simulink model "integrated_controller_scenario3"  (R2021a)
settings: Solver=VariableStepAuto  StartTime=0.0  StopTime=50  RelTol=1e-3
values from neighbouring files (symbols this model uses):
  Cf = 155494.663    [integrated_controller_init.m]    (also in integrated_controller_init_q3.m; integrated_controller_init_q4.m; integrated_controller_init_q5.m; integrated_controller_init_q6_MRM.m)
  Cr = 1554494.663    [integrated_controller_init.m]    (also in integrated_controller_init_q3.m; integrated_controller_init_q4.m; integrated_controller_init_q5.m; integrated_controller_init_q6_MRM.m)
  Iz = 1436.24    [integrated_controller_init.m]    (also in integrated_controller_init_q3.m; integrated_controller_init_q4.m; integrated_controller_init_q5.m; integrated_controller_init_q6_MRM.m)
  L = 3.5    [alc_pathplanning.m]    (also in integrated_controller_init.m = 4.7; integrated_controller_init_q3.m = 4.7; integrated_controller_init_q4.m = 4.7; integrated_controller_init_q5.m = 4.7)
  ld = 10    [integrated_controller_init.m]    (also in integrated_controller_init_q3.m; integrated_controller_init_q4.m; integrated_controller_init_q5.m; integrated_controller_init_q6_MRM.m)
  lf = 1.165    [integrated_controller_init.m]    (also in integrated_controller_init_q3.m; integrated_controller_init_q4.m; integrated_controller_init_q5.m; integrated_controller_init_q6_MRM.m)
  lr = 1.165    [integrated_controller_init.m]    (also in integrated_controller_init_q3.m; integrated_controller_init_q4.m; integrated_controller_init_q5.m; integrated_controller_init_q6_MRM.m)
  m = 1140    [integrated_controller_init.m]    (also in integrated_controller_init_q3.m; integrated_controller_init_q4.m; integrated_controller_init_q5.m; integrated_controller_init_q6_MRM.m)
  md = get_curvature(Vx,yaw_rate_pose,tRef')    [integrated_controller_init.m]    (also in integrated_controller_init_q3.m; integrated_controller_init_q4.m; integrated_controller_init_q5.m; integrated_controller_init_q6_MRM.m)
  Ts = 0.1    [integrated_controller_init.m]    (also in integrated_controller_init_q3.m; integrated_controller_init_q4.m; integrated_controller_init_q5.m; integrated_controller_init_q6_MRM.m)
  V_initial = 15    [integrated_controller_init.m]    (also in integrated_controller_init_q3.m = 11; integrated_controller_init_q4.m = 25; integrated_controller_init_q5.m; integrated_controller_init_q6_MRM.m)
  Vx = a(2) + 2*a(3)*t + 3*a(4)*t.^2 +4*a(5)*t.^3+ a(6)*t.^4    [alc_pathplanning.m]    (also in integrated_controller_init.m = 18; integrated_controller_init_q3.m = 20; integrated_controller_init_q4.m = 25; integrated_controller_init_q5.m = 15)
  xRef = X_ref    [alc_pathplanning.m]    (also in integrated_controller_init.m = path.xRef; integrated_controller_init_q3.m = path.xRef; integrated_controller_init_q4.m = path.xRef; integrated_controller_init_q5.m = refPose(1,:))
  yRef = Y_ref    [alc_pathplanning.m]    (also in integrated_controller_init.m = path.yRef; integrated_controller_init_q3.m = path.yRef; integrated_controller_init_q4.m = path.yRef; integrated_controller_init_q5.m = refPose(2,:))
undefined symbols (not defined in the file or in its folder): sigbuilder_block
libraries: pid_lib x2, mpcadaslib x1, robotalgslib x1, autolibshared x1
settings Model: Creator=anime  LastModifiedBy=srini
settings SolverCC: AlgebraicLoopSolver=TrustRegion
settings DebuggingCC: SFMachineParentedDataDiag=warning

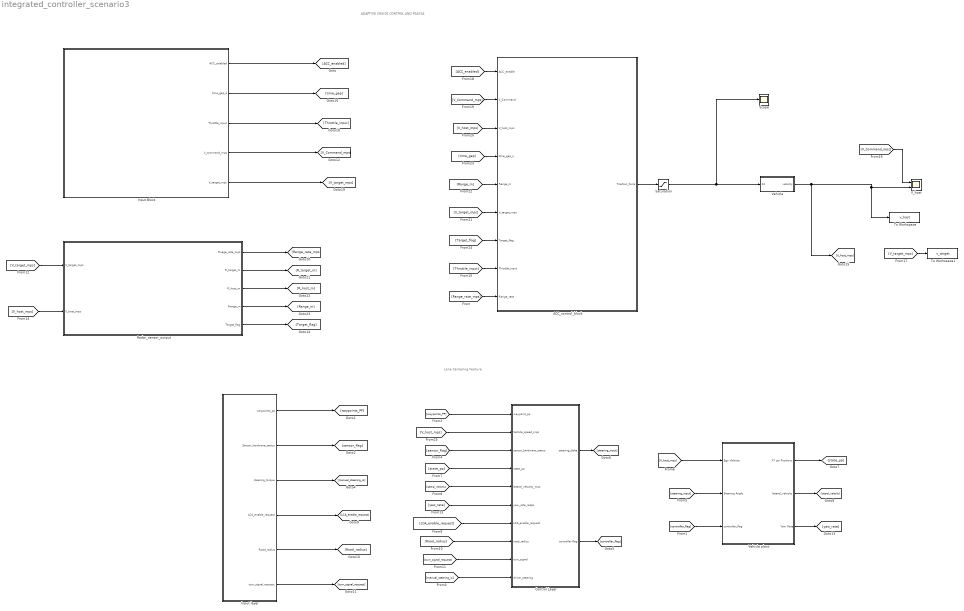
== system integrated_controller_scenario3 ==
  note: ADAPTIVE CRUISE CONTROL AND PSA/ISA
  note: Lane Centering Feature
  ACC_control_block : Subsystem
  Control Layer : Subsystem
  Input Block : Subsystem
  Input layer : Subsystem
  Radar_sensor_output : Subsystem
  Saturation : Saturate  UpperLimit=1000  LowerLimit=-1000  ZeroCross=off
  Scope : Scope
  To Workspace : ToWorkspace  VariableName=v_host  SaveFormat=Timeseries  SampleTime=-1
  To Workspace1 : ToWorkspace  VariableName=v_target  SaveFormat=Timeseries  SampleTime=-1
  V_host : Scope  NumInputPorts=2
  Vehicle : Subsystem
  Vehicle plant : Subsystem
  wires:
  Vehicle plant/3(Yaw Rate) -> [yaw_rate]
  [yaw_rate] -> Control Layer/6(yaw_rate_radps)
  Vehicle plant/2(lateral_velocity) -> [lateral_velocity]
  [lateral_velocity] -> Control Layer/5(lateral_velocity_mps)
  Input layer/2(Sensor_hardware_status) -> [sensor_flag]
  [turn_signal_request] -> Control Layer/9(turn_signal)
  Control Layer/2(controller flag) -> [controller_flag]
  [controller_flag] -> Vehicle plant/3(controller_flag)
  [steering_input] -> Vehicle plant/2(Steering Angle)
  Input layer/5(Road_radius) -> [Road_radius]
  Input layer/1(waypoints_pp) -> [waypoints_PP]
  [LCA_enable_request] -> Control Layer/7(LCA_enable_request)
  [sensor_flag] -> Control Layer/3(sensor_hardware_status)
  Input layer/4(LCA_enable_request) -> [LCA_enable_request]
  Vehicle plant/1(XY psi Positions) -> [state_pp]
  Input layer/6(turn_signal_request) -> [turn_signal_request]
  Input layer/3(steering_torque) -> [manual_steering_io]
  [manual_steering_io] -> Control Layer/10(driver_steering)
  [waypoints_PP] -> Control Layer/1(waypoint_pp)
  Control Layer/1(steering_delta) -> [steering_input]
  [state_pp] -> Control Layer/4(state_pp)
  [Road_radius] -> Control Layer/8(road_radius)
  [Range_m] -> ACC_control_block/5(Range_m)
  ACC_control_block/1(Traction_force) -> Saturation/1
  [Throttle_input] -> ACC_control_block/8(Throttle_input)
  [V_Command_mps] -> ACC_control_block/2(V_Command)
  [ACC_enabled] -> ACC_control_block/1(ACC_enable)
  [time_gap] -> ACC_control_block/4(time_gap_s)
  Vehicle/1(velocity) -> [V_host_mps], To Workspace/1, V_host/2
  [V_host_mps] -> ACC_control_block/3(V_host_mps)
  Radar_sensor_output/5(Target_flag) -> [Target_flag]
  [Target_flag] -> ACC_control_block/7(Target_flag)
  [V_target_mps] -> ACC_control_block/6(V_target_mps)
  Radar_sensor_output/3(R_host_m) -> [R_host_m]
  Input Block/4(" V_command_mps") -> [V_Command_mps]
  [V_Command_mps] -> V_host/1
  [V_target_mps] -> Radar_sensor_output/1(V_target_mps)
  Input Block/2(" time_gap_s") -> [time_gap]
  Input Block/5(" V_target_mps") -> [V_target_mps]
  [V_host_mps] -> Radar_sensor_output/2(V_host_mps)
  Radar_sensor_output/1(Rnage_rate_mps) -> [Range_rate_mps]
  Input Block/3(" Throttle_input") -> [Throttle_input]
  Radar_sensor_output/2(R_target_m) -> [R_target_m]
  Radar_sensor_output/4(Range_m) -> [Range_m]
  [V_target_mps] -> To Workspace1/1
  Input Block/1(" ACC_enabled") -> [ACC_enabled]
  [V_host_mps] -> Control Layer/2(Vehicle_speed_mps)
  [Range_rate_mps] -> ACC_control_block/9(Range_rate)
  Saturation/1 -> Scope/1, Vehicle/1(Fd)
  [V_host_mps] -> Vehicle plant/1(Ego Velocity)

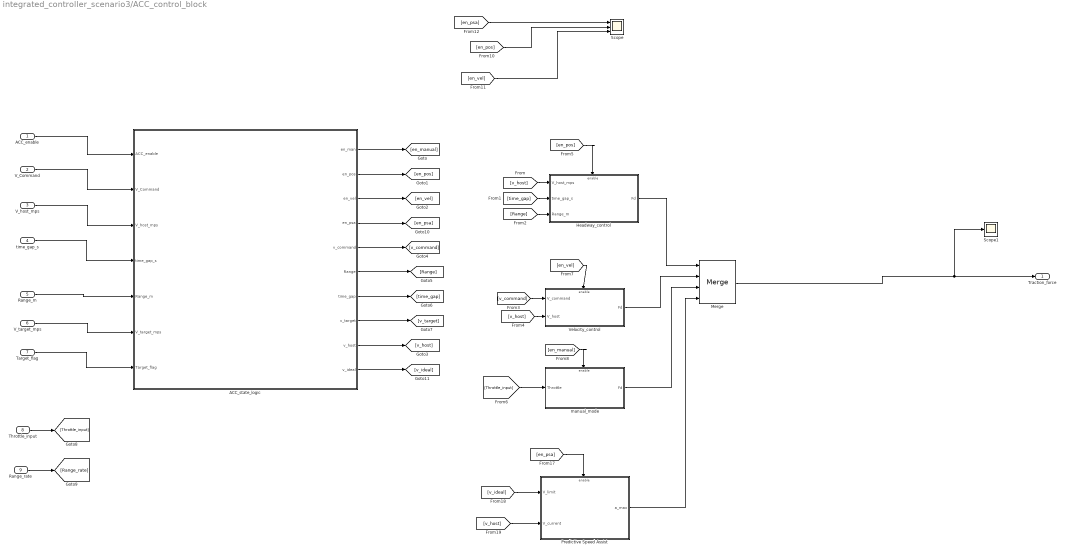
== system integrated_controller_scenario3/ACC_control_block ==
  ACC_enable : Inport
  V_Command : Inport  Port=2
  V_host_mps : Inport  Port=3
  time_gap_s : Inport  Port=4
  Range_m : Inport  Port=5
  V_target_mps : Inport  Port=6
  Target_flag : Inport  Port=7
  Throttle_input : Inport  Port=8
  Range_rate : Inport  Port=9
  ACC_state_logic : Subsystem
  Headway_control : Subsystem
  Merge : Merge  Inputs=4
  "Predictive Speed Assist " : Subsystem  TreatAsAtomicUnit=on
  Scope : Scope  NumInputPorts=3
  Scope1 : Scope
  Velocity_control : Subsystem
  manual_mode : Subsystem
  Traction_force : Outport
  wires:
  ACC_enable/1 -> ACC_state_logic/1(ACC_enable)
  V_Command/1 -> ACC_state_logic/2(V_Command)
  V_host_mps/1 -> ACC_state_logic/3(V_host_mps)
  time_gap_s/1 -> ACC_state_logic/4(time_gap_s)
  Range_m/1 -> ACC_state_logic/5(Range_m)
  V_target_mps/1 -> ACC_state_logic/6(V_target_mps)
  Target_flag/1 -> ACC_state_logic/7(Target_flag)
  ACC_state_logic/1(en_man) -> [en_manual]
  ACC_state_logic/2(en_pos) -> [en_pos]
  ACC_state_logic/3(en_vel) -> [en_vel]
  ACC_state_logic/9(v_host) -> [v_host]
  ACC_state_logic/5(v_command) -> [v_command]
  ACC_state_logic/6(Range) -> [Range]
  ACC_state_logic/7(time_gap) -> [time_gap]
  ACC_state_logic/8(v_target) -> [v_target]
  [v_host] -> Headway_control/1(V_host_mps)
  [time_gap] -> Headway_control/2(time_gap_s)
  [Range] -> Headway_control/3(Range_m)
  [v_command] -> Velocity_control/1(V_command)
  [v_host] -> Velocity_control/2(V_host)
  [en_pos] -> Headway_control/Enable
  Throttle_input/1 -> [Throttle_input]
  [Throttle_input] -> manual_mode/1(Throttle)
  [en_vel] -> Velocity_control/Enable
  [en_manual] -> manual_mode/Enable
  Headway_control/1(Fd) -> Merge/1
  Velocity_control/1(Fd) -> Merge/2
  manual_mode/1(Fd) -> Merge/3
  [en_pos] -> Scope/2
  [en_vel] -> Scope/3
  Range_rate/1 -> [Range_rate]
  ACC_state_logic/4(en_psa) -> [en_psa]
  [en_psa] -> "Predictive Speed Assist "/Enable
  ACC_state_logic/10(v_ideal) -> [v_ideal]
  [v_ideal] -> "Predictive Speed Assist "/1(V_limit)
  [v_host] -> "Predictive Speed Assist "/2(V_current)
  "Predictive Speed Assist "/1(a_max) -> Merge/4
  Merge/1 -> Scope1/1, Traction_force/1
  [en_psa] -> Scope/1

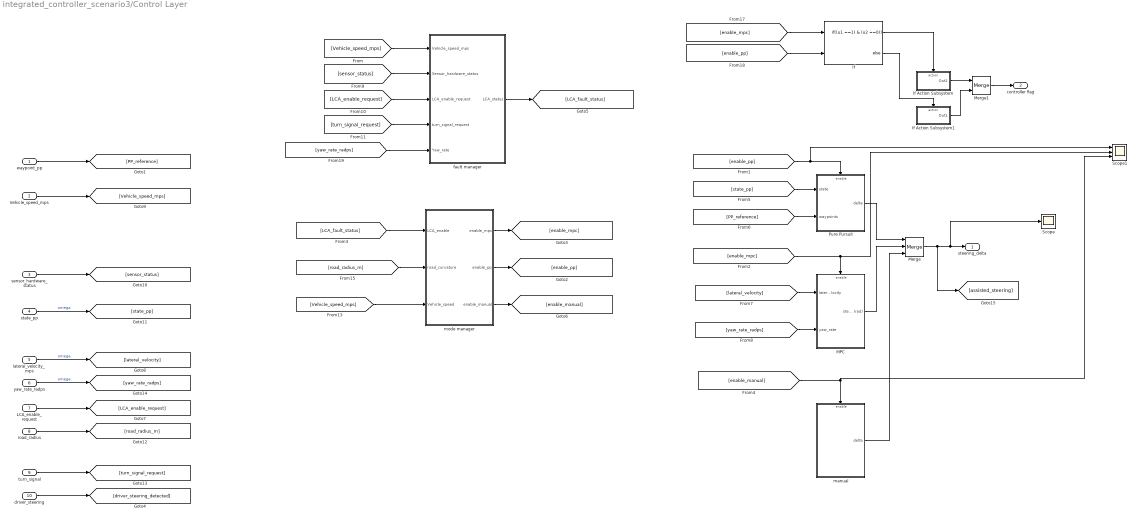
== system integrated_controller_scenario3/Control Layer ==
  waypoint_pp : Inport
  Vehicle_speed_mps : Inport  Port=2
  sensor_hardware_status : Inport  Port=3
  state_pp : Inport  Port=4
  lateral_velocity_mps : Inport  Port=5
  yaw_rate_radps : Inport  Port=6
  LCA_enable_request : Inport  Port=7
  road_radius : Inport  Port=8
  turn_signal : Inport  Port=9
  driver_steering : Inport  Port=10
  If : If  NumInputs=2  IfExpression=(u1 ==1) & (u2 ==0)
  If Action Subsystem : Subsystem  TreatAsAtomicUnit=on
  If Action Subsystem1 : Subsystem  TreatAsAtomicUnit=on
  MPC : Subsystem
  Merge : Merge  Inputs=3
  Merge1 : Merge
  Pure Pursuit : Subsystem
  Scope : Scope
  Scope1 : Scope  NumInputPorts=3
  fault manager : Subsystem
  manual : Subsystem
  mode manager : Subsystem
  steering_delta : Outport
  controller flag : Outport  Port=2
  wires:
  [Vehicle_speed_mps] -> fault manager/1(Vehicle_speed_mps)
  fault manager/1(LCA_status) -> [LCA_fault_status]
  [enable_pp] -> Scope1/1, Pure Pursuit/Enable
  [road_radius_m] -> mode manager/2(road_curvature)
  Pure Pursuit/1(delta) -> Merge/1
  MPC/1(steering angle (rad)) -> Merge/2
  Merge/1 -> [assisted_steering], Scope/1, steering_delta/1
  [state_pp] -> Pure Pursuit/1(state)
  [PP_reference] -> Pure Pursuit/2(waypoints)
  waypoint_pp/1 -> [PP_reference]
  Vehicle_speed_mps/1 -> [Vehicle_speed_mps]
  sensor_hardware_status/1 -> [sensor_status]
  state_pp/1 -> [state_pp]  "omega"
  lateral_velocity_mps/1 -> [lateral_velocity]  "omega"
  LCA_enable_request/1 -> [LCA_enable_request]
  [sensor_status] -> fault manager/2(Sensor_hardware_status)
  [LCA_enable_request] -> fault manager/3(LCA_enable_request)
  [Vehicle_speed_mps] -> mode manager/3(Vehicle_speed)
  mode manager/2(enable_pp) -> [enable_pp]
  mode manager/1(enable_mpc) -> [enable_mpc]
  road_radius/1 -> [road_radius_m]
  [LCA_fault_status] -> mode manager/1(LCA_enable)
  mode manager/3(enable_manual) -> [enable_manual]
  [enable_manual] -> Scope1/3, manual/Enable
  manual/1(delta) -> Merge/3
  turn_signal/1 -> [turn_signal_request]
  [turn_signal_request] -> fault manager/4(turn_signal_request)
  [enable_mpc] -> Scope1/2, MPC/Enable
  yaw_rate_radps/1 -> [yaw_rate_radps]  "omega"
  [lateral_velocity] -> MPC/1(lateral_velocity)
  [yaw_rate_radps] -> MPC/2(yaw_rate)
  driver_steering/1 -> [driver_steering_detected]
  [enable_mpc] -> If/1
  [enable_pp] -> If/2
  If/1 -> If Action Subsystem/Action
  If Action Subsystem/1(Out1) -> Merge1/1
  Merge1/1 -> controller flag/1
  If/2 -> If Action Subsystem1/Action
  If Action Subsystem1/1(Out1) -> Merge1/2
  [yaw_rate_radps] -> fault manager/5(Yaw_rate)

== system integrated_controller_scenario3/Input Block ==
  Constant : Constant  Value=8
  Set_speed : Constant  Value=Vx
  Signal Builder : Subsystem  Tag=STV Subsys  LoadFcn=sigbuilder_block('load');  StartFcn=sigbuilder_block('start');  StopFcn=sigbuilder_block('stop');  ClipboardFcn=sigbuilder_block('clipboard');  mask(Sigbuilder block){tuvar=[0:10]}
      mask help: Simulink:masks:SigbuilderBlock_MD
      mask init:
      | if ~strcmp(get_param(bdroot(gcbh),'SimulationStatus'),'stopped') tuvar = sigbuilder_block('maskInit'); end
      settings: CopyFcn=sigbuilder_block('copy');  DeleteFcn=sigbuilder_block('delete');  ModelCloseFcn=sigbuilder_block('modelClose');  PreSaveFcn=sigbuilder_block('preSave');  PauseFcn=sigbuilder_block('pause');  ContinueFcn=sigbuilder_block('continue');  NameChangeFcn=sigbuilder_block('namechange');  OpenFcn=sigbuilder_block('open',[969.75 323.25 944.25 311.25 ]);  CloseFcn=sigbuilder_block('close');
      mask Display: plot(0, 0, 100, 100,[2, 2, 32, 32, 2], [68, 8, 8, 68, 68],[32, 2], [38, 38], [32, 19, 2],[53, 60, 44], [32, 17, 17, 2],[16, 16, 31, 31]);txt = getActiveGroup(gcbh);text(2, 100, txt,'verticalAlignment', 'top');
  Throttle : Constant  Value=0
  time_gap : Constant  Value=4
  " ACC_enabled" : Outport
  " time_gap_s" : Outport  Port=2
  " Throttle_input" : Outport  Port=3
  " V_command_mps" : Outport  Port=4
  " V_target_mps" : Outport  Port=5
  wires:
  time_gap/1 -> " time_gap_s"/1
  Throttle/1 -> " Throttle_input"/1
  Set_speed/1 -> " V_command_mps"/1
  Constant/1 -> " V_target_mps"/1
  Signal Builder/1(ACC_Enable_1) -> " ACC_enabled"/1

== system integrated_controller_scenario3/Input layer ==
  LCA_enable_request_signal : Subsystem  Tag=STV Subsys  LoadFcn=sigbuilder_block('load');  StartFcn=sigbuilder_block('start');  StopFcn=sigbuilder_block('stop');  ClipboardFcn=sigbuilder_block('clipboard');  mask(Sigbuilder block){tuvar=[0:10]}
      mask help: Simulink:masks:SigbuilderBlock_MD
      mask init:
      | if ~strcmp(get_param(bdroot(gcbh),'SimulationStatus'),'stopped') tuvar = sigbuilder_block('maskInit'); end
      settings: CopyFcn=sigbuilder_block('copy');  DeleteFcn=sigbuilder_block('delete');  ModelCloseFcn=sigbuilder_block('modelClose');  PreSaveFcn=sigbuilder_block('preSave');  PauseFcn=sigbuilder_block('pause');  ContinueFcn=sigbuilder_block('continue');  NameChangeFcn=sigbuilder_block('namechange');  OpenFcn=sigbuilder_block('open',[437.6 199.2 550.4 400 ]);  CloseFcn=sigbuilder_block('close');
      mask Display: plot(0, 0, 100, 100,[2, 2, 32, 32, 2], [68, 8, 8, 68, 68],[32, 2], [38, 38], [32, 19, 2],[53, 60, 44], [32, 17, 17, 2],[16, 16, 31, 31]);txt = getActiveGroup(gcbh);text(2, 100, txt,'verticalAlignment', 'top');
  Reference for PP : Subsystem
  Road_radius_signal : Subsystem  Tag=STV Subsys  LoadFcn=sigbuilder_block('load');  StartFcn=sigbuilder_block('start');  StopFcn=sigbuilder_block('stop');  ClipboardFcn=sigbuilder_block('clipboard');  mask(Sigbuilder block){tuvar=[0:10]}
      mask help: Simulink:masks:SigbuilderBlock_MD
      mask init:
      | if ~strcmp(get_param(bdroot(gcbh),'SimulationStatus'),'stopped') tuvar = sigbuilder_block('maskInit'); end
      settings: CopyFcn=sigbuilder_block('copy');  DeleteFcn=sigbuilder_block('delete');  ModelCloseFcn=sigbuilder_block('modelClose');  PreSaveFcn=sigbuilder_block('preSave');  PauseFcn=sigbuilder_block('pause');  ContinueFcn=sigbuilder_block('continue');  NameChangeFcn=sigbuilder_block('namechange');  OpenFcn=sigbuilder_block('open',[437.6 199.2 550.4 400 ]);  CloseFcn=sigbuilder_block('close');
      mask Display: plot(0, 0, 100, 100,[2, 2, 32, 32, 2], [68, 8, 8, 68, 68],[32, 2], [38, 38], [32, 19, 2],[53, 60, 44], [32, 17, 17, 2],[16, 16, 31, 31]);txt = getActiveGroup(gcbh);text(2, 100, txt,'verticalAlignment', 'top');
  sensor fault status : Subsystem  Tag=STV Subsys  LoadFcn=sigbuilder_block('load');  StartFcn=sigbuilder_block('start');  StopFcn=sigbuilder_block('stop');  ClipboardFcn=sigbuilder_block('clipboard');  mask(Sigbuilder block){tuvar=[0:10]}
      mask help: Simulink:masks:SigbuilderBlock_MD
      mask init:
      | if ~strcmp(get_param(bdroot(gcbh),'SimulationStatus'),'stopped') tuvar = sigbuilder_block('maskInit'); end
      settings: CopyFcn=sigbuilder_block('copy');  DeleteFcn=sigbuilder_block('delete');  ModelCloseFcn=sigbuilder_block('modelClose');  PreSaveFcn=sigbuilder_block('preSave');  PauseFcn=sigbuilder_block('pause');  ContinueFcn=sigbuilder_block('continue');  NameChangeFcn=sigbuilder_block('namechange');  OpenFcn=sigbuilder_block('open',[437.6 199.2 550.4 400 ]);  CloseFcn=sigbuilder_block('close');
      mask Display: plot(0, 0, 100, 100,[2, 2, 32, 32, 2], [68, 8, 8, 68, 68],[32, 2], [38, 38], [32, 19, 2],[53, 60, 44], [32, 17, 17, 2],[16, 16, 31, 31]);txt = getActiveGroup(gcbh);text(2, 100, txt,'verticalAlignment', 'top');
  steering_torque_signal : Subsystem  Tag=STV Subsys  LoadFcn=sigbuilder_block('load');  StartFcn=sigbuilder_block('start');  StopFcn=sigbuilder_block('stop');  ClipboardFcn=sigbuilder_block('clipboard');  mask(Sigbuilder block){tuvar=[0:10]}
      mask help: Simulink:masks:SigbuilderBlock_MD
      mask init:
      | if ~strcmp(get_param(bdroot(gcbh),'SimulationStatus'),'stopped') tuvar = sigbuilder_block('maskInit'); end
      settings: CopyFcn=sigbuilder_block('copy');  DeleteFcn=sigbuilder_block('delete');  ModelCloseFcn=sigbuilder_block('modelClose');  PreSaveFcn=sigbuilder_block('preSave');  PauseFcn=sigbuilder_block('pause');  ContinueFcn=sigbuilder_block('continue');  NameChangeFcn=sigbuilder_block('namechange');  OpenFcn=sigbuilder_block('open',[437.6 199.2 550.4 400 ]);  CloseFcn=sigbuilder_block('close');
      mask Display: plot(0, 0, 100, 100,[2, 2, 32, 32, 2], [68, 8, 8, 68, 68],[32, 2], [38, 38], [32, 19, 2],[53, 60, 44], [32, 17, 17, 2],[16, 16, 31, 31]);txt = getActiveGroup(gcbh);text(2, 100, txt,'verticalAlignment', 'top');
  turn_signal : Subsystem  Tag=STV Subsys  LoadFcn=sigbuilder_block('load');  StartFcn=sigbuilder_block('start');  StopFcn=sigbuilder_block('stop');  ClipboardFcn=sigbuilder_block('clipboard');  mask(Sigbuilder block){tuvar=[0:10]}
      mask help: Simulink:masks:SigbuilderBlock_MD
      mask init:
      | if ~strcmp(get_param(bdroot(gcbh),'SimulationStatus'),'stopped') tuvar = sigbuilder_block('maskInit'); end
      settings: CopyFcn=sigbuilder_block('copy');  DeleteFcn=sigbuilder_block('delete');  ModelCloseFcn=sigbuilder_block('modelClose');  PreSaveFcn=sigbuilder_block('preSave');  PauseFcn=sigbuilder_block('pause');  ContinueFcn=sigbuilder_block('continue');  NameChangeFcn=sigbuilder_block('namechange');  OpenFcn=sigbuilder_block('open',[437.6 199.2 550.4 400 ]);  CloseFcn=sigbuilder_block('close');
      mask Display: plot(0, 0, 100, 100,[2, 2, 32, 32, 2], [68, 8, 8, 68, 68],[32, 2], [38, 38], [32, 19, 2],[53, 60, 44], [32, 17, 17, 2],[16, 16, 31, 31]);txt = getActiveGroup(gcbh);text(2, 100, txt,'verticalAlignment', 'top');
  waypoints_pp : Outport
  Sensor_hardware_status : Outport  Port=2
  steering_torque : Outport  Port=3
  LCA_enable_request : Outport  Port=4
  Road_radius : Outport  Port=5
  turn_signal_request : Outport  Port=6
  wires:
  Reference for PP/1(Waypoints) -> waypoints_pp/1
  sensor fault status/1(Signal 1) -> Sensor_hardware_status/1
  steering_torque_signal/1(Signal 1) -> steering_torque/1
  LCA_enable_request_signal/1(Signal 2) -> LCA_enable_request/1
  Road_radius_signal/1(Signal 2) -> Road_radius/1
  turn_signal/1(Signal 2) -> turn_signal_request/1

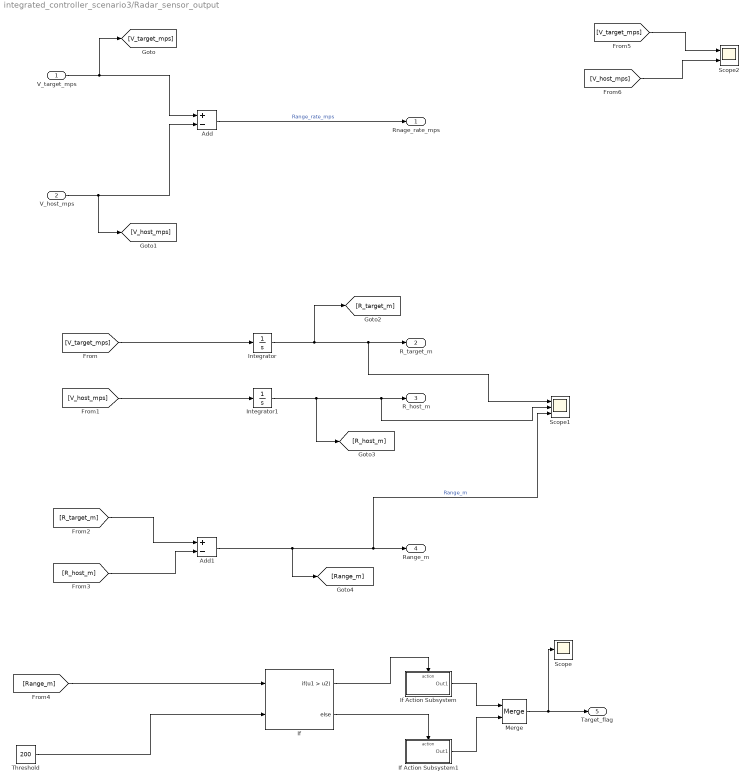
== system integrated_controller_scenario3/Radar_sensor_output ==
  V_target_mps : Inport
  V_host_mps : Inport  Port=2
  Add : Sum  Inputs=+-
  Add1 : Sum  Inputs=+-
  If : If  NumInputs=2  IfExpression=u1 > u2
  If Action Subsystem : Subsystem  TreatAsAtomicUnit=on
  If Action Subsystem1 : Subsystem  TreatAsAtomicUnit=on
  Integrator : Integrator  InitialCondition=200000
  Integrator1 : Integrator
  Merge : Merge
  Scope : Scope
  Scope1 : Scope  NumInputPorts=3
  Scope2 : Scope  NumInputPorts=2
  Threshold : Constant  Value=200
  Rnage_rate_mps : Outport
  R_target_m : Outport  Port=2
  R_host_m : Outport  Port=3
  Range_m : Outport  Port=4
  Target_flag : Outport  Port=5
  wires:
  V_target_mps/1 -> [V_target_mps], Add/1
  V_host_mps/1 -> [V_host_mps], Add/2
  Add/1 -> Rnage_rate_mps/1  "Range_rate_mps"
  Integrator/1 -> [R_target_m], Scope1/1, R_target_m/1
  [V_target_mps] -> Integrator/1
  [V_host_mps] -> Integrator1/1
  Integrator1/1 -> [R_host_m], Scope1/2, R_host_m/1
  [R_target_m] -> Add1/1
  [R_host_m] -> Add1/2
  Add1/1 -> [Range_m], Scope1/3, Range_m/1  "Range_m"
  [Range_m] -> If/1
  Threshold/1 -> If/2
  If/1 -> If Action Subsystem/Action
  If/2 -> If Action Subsystem1/Action
  If Action Subsystem/1(Out1) -> Merge/1
  If Action Subsystem1/1(Out1) -> Merge/2
  Merge/1 -> Scope/1, Target_flag/1
  [V_target_mps] -> Scope2/1
  [V_host_mps] -> Scope2/2

== system integrated_controller_scenario3/Vehicle ==
  Fd : Inport
  Gain : Gain  Gain=9.211*1e-4
  Gain1 : Gain  Gain=0.0216
  Integrator : Integrator  InitialCondition=V_initial
  Sum : Sum  Inputs=|+-
  velocity : Outport
  wires:
  Integrator/1 -> Gain1/1, velocity/1
  Gain/1 -> Sum/1
  Fd/1 -> Gain/1  "Input_u"
  Gain1/1 -> Sum/2
  Sum/1 -> Integrator/1

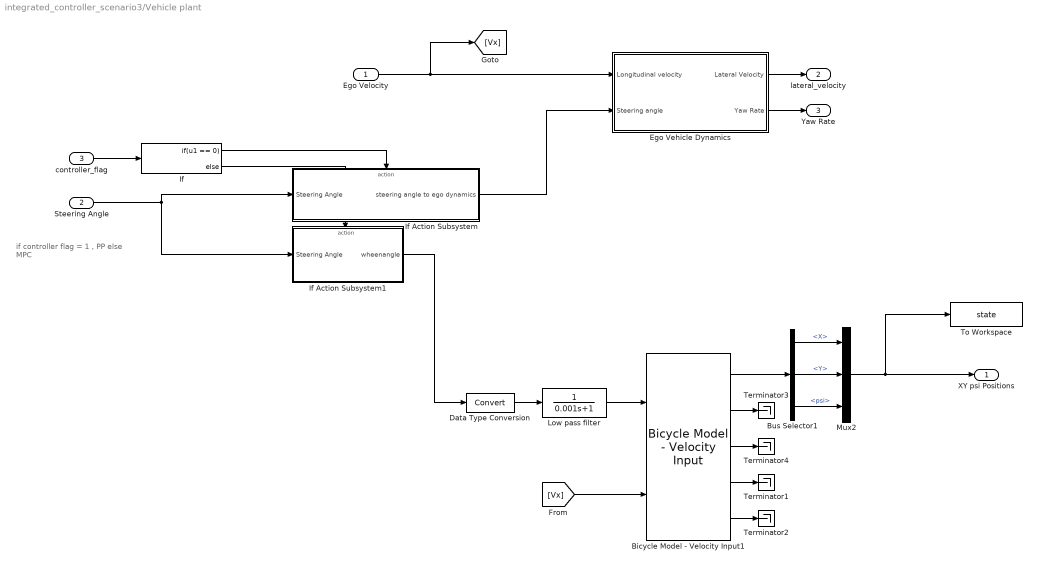
== system integrated_controller_scenario3/Vehicle plant ==
  note: if controller flag = 1 , PP
      | else MPC
  Ego Velocity : Inport
  Steering Angle : Inport  Port=2
  controller_flag : Inport  Port=3
  Bicycle Model - Velocity Input1 : autolibshared/Bicycle Model - Velocity Input  trackMode=Single (bicycle)  inputMode=External longitudinal forces  frontSteerMode=on  rearSteerMode=off  windMode=off  muMode=off  extFMode=off  extMMode=off  aMode=3  NF=2  NR=2  m=m  a=lf  b=lr  h=0.35  X_o=X_o  xdot_o=0  CalphaMode=off  sigmaMode=on  w=[1.4,1.4]  Cy_f=Cf  Cy_r=Cr  sigma_f=.1  sigma_r=.1  alpha_f_brk=[-.1 .1]  Cy_f_data=[-9e3 9e3]  alpha_r_brk=[-.1 .1]  Cy_r_data=[-9e3 9e3]  Y_o=Y_o  ydot_o=0  Izz=Iz  psi_o=0  r_o=0  Af=2  Cd=.3  Cl=.1  Cpm=.1  beta_w=[0:0.01:0.3]  Cs=[0:0.03:0.9]  Cym=[0:0.01:0.3]  Pabs=101325  Tair=273  g=9.81  mu=1  xdot_tol=.01  Fznom=5000  Fxtire_sat=1e6  Fytire_sat=1e6  longOff=0  latOff=0  vertOff=0
      settings: SourceProductBaseCode=PW,DR,MT,UV,VE
  Bus Selector1 : BusSelector  OutputSignals=InertFrm.FrntAxl.Disp.X,InertFrm.FrntAxl.Disp.Y,InertFrm.Cg.Ang.psi
  Data Type Conversion : DataTypeConversion
  Ego Vehicle Dynamics : Subsystem
  If : If  IfExpression=u1 == 0
  If Action Subsystem : Subsystem  TreatAsAtomicUnit=on
  If Action Subsystem1 : Subsystem  TreatAsAtomicUnit=on
  Low pass filter : TransferFcn  Denominator=[0.001 1]
  Mux2 : Mux  Inputs=3
  Terminator{1..4} (4 alike) : Terminator
  To Workspace : ToWorkspace  VariableName=state  SampleTime=-1
  XY psi Positions : Outport  Unit=m  VectorParamsAs1DForOutWhenUnconnected=off
  lateral_velocity : Outport  Port=2  Unit=m/s  VectorParamsAs1DForOutWhenUnconnected=off
  Yaw Rate : Outport  Port=3  Unit=degree/s  VectorParamsAs1DForOutWhenUnconnected=off
  wires:
  Bicycle Model - Velocity Input1/3 -> Terminator4/1
  Bicycle Model - Velocity Input1/2 -> Terminator3/1
  Data Type Conversion/1 -> Low pass filter/1
  Mux2/1 -> To Workspace/1, XY psi Positions/1
  Bicycle Model - Velocity Input1/1 -> Bus Selector1/1
  Low pass filter/1 -> Bicycle Model - Velocity Input1/1
  Bicycle Model - Velocity Input1/5 -> Terminator2/1
  Bus Selector1/1 -> Mux2/1  "<X>"
  Bus Selector1/2 -> Mux2/2  "<Y>"
  Bicycle Model - Velocity Input1/4 -> Terminator1/1
  Bus Selector1/3 -> Mux2/3  "<psi>"
  Ego Velocity/1 -> [Vx], Ego Vehicle Dynamics/1(Longitudinal velocity)
  Ego Vehicle Dynamics/2(Yaw Rate) -> Yaw Rate/1
  Ego Vehicle Dynamics/1(Lateral Velocity) -> lateral_velocity/1
  [Vx] -> Bicycle Model - Velocity Input1/2
  controller_flag/1 -> If/1
  Steering Angle/1 -> If Action Subsystem1/1(Steering Angle), If Action Subsystem/1(Steering Angle)
  If/1 -> If Action Subsystem/Action
  If/2 -> If Action Subsystem1/Action
  If Action Subsystem/1(steering angle to ego dynamics) -> Ego Vehicle Dynamics/2(Steering angle)
  If Action Subsystem1/1(wheenangle) -> Data Type Conversion/1

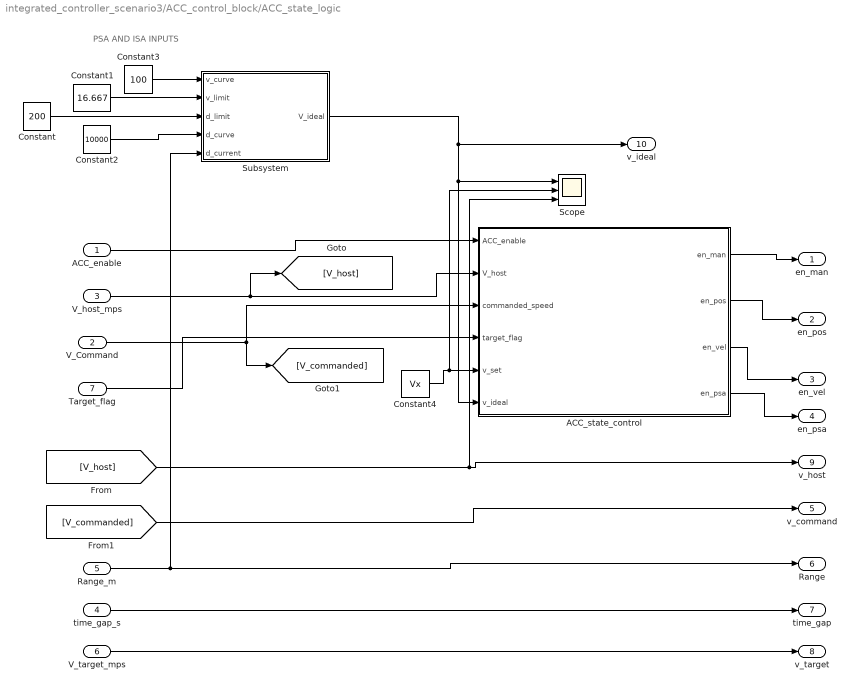
== system integrated_controller_scenario3/ACC_control_block/ACC_state_logic ==
  note: PSA AND ISA INPUTS
  ACC_enable : Inport
  V_Command : Inport  Port=2
  V_host_mps : Inport  Port=3
  time_gap_s : Inport  Port=4
  Range_m : Inport  Port=5
  V_target_mps : Inport  Port=6
  Target_flag : Inport  Port=7
  ACC_state_control : Stateflow chart  TreatAsAtomicUnit=on
  Constant : Constant  Value=200
  Constant1 : Constant  Value=16.667
  Constant2 : Constant  Value=10000
  Constant3 : Constant  Value=100
  Constant4 : Constant  Value=Vx
  Scope : Scope  NumInputPorts=3
  Subsystem : Subsystem
  en_man : Outport
  en_pos : Outport  Port=2
  en_vel : Outport  Port=3
  en_psa : Outport  Port=4
  v_command : Outport  Port=5
  Range : Outport  Port=6
  time_gap : Outport  Port=7
  v_target : Outport  Port=8
  v_host : Outport  Port=9
  v_ideal : Outport  Port=10
  wires:
  ACC_enable/1 -> ACC_state_control/1(ACC_enable)
  V_Command/1 -> [V_commanded], ACC_state_control/3(commanded_speed)
  V_host_mps/1 -> [V_host], ACC_state_control/2(V_host)
  Target_flag/1 -> ACC_state_control/4(target_flag)
  ACC_state_control/1(en_man) -> en_man/1
  ACC_state_control/2(en_pos) -> en_pos/1
  ACC_state_control/3(en_vel) -> en_vel/1
  [V_host] -> Scope/3, v_host/1
  [V_commanded] -> v_command/1
  Range_m/1 -> Subsystem/5(d_current), Range/1
  time_gap_s/1 -> time_gap/1
  V_target_mps/1 -> v_target/1
  Subsystem/1(V_ideal) -> v_ideal/1, ACC_state_control/6(v_ideal), Scope/1
  ACC_state_control/4(en_psa) -> en_psa/1
  Constant/1 -> Subsystem/3(d_limit)
  Constant1/1 -> Subsystem/2(v_limit)
  Constant2/1 -> Subsystem/4(d_curve)
  Constant3/1 -> Subsystem/1(v_curve)
  Constant4/1 -> Scope/2, ACC_state_control/5(v_set)

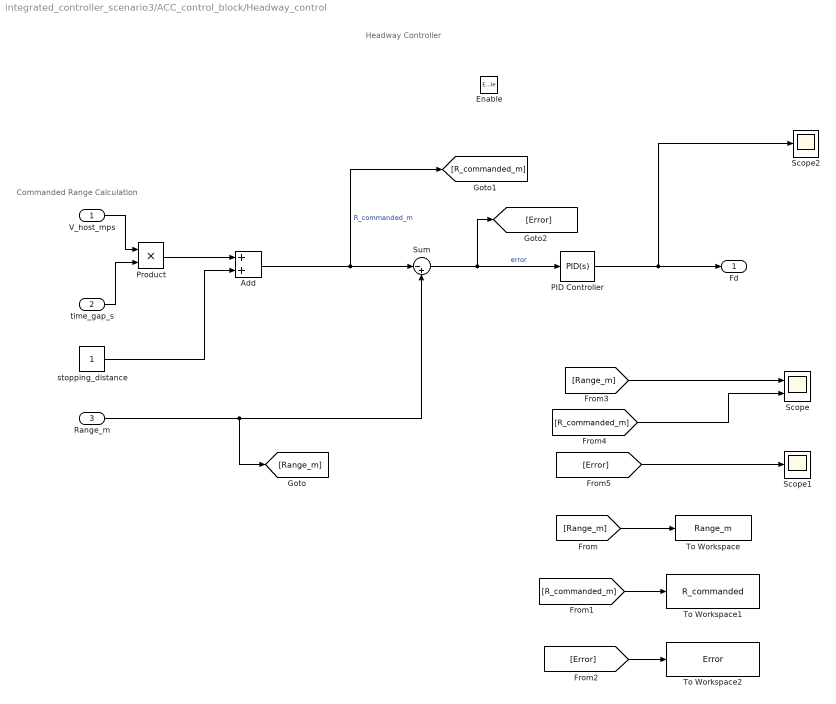
== system integrated_controller_scenario3/ACC_control_block/Headway_control ==
  note: Headway Controller
  note: Commanded Range Calculation
  V_host_mps : Inport
  time_gap_s : Inport  Port=2
  Range_m : Inport  Port=3
  Enable : EnablePort
  Add : Sum
  PID Controller : pid_lib/PID Controller  Controller=PID  Form=Parallel  TimeDomain=Continuous-time  UseExternalTs=off  SampleTime=-1  IntegratorMethod=Forward Euler  FilterMethod=Forward Euler  ControllerParametersSource=internal  P=1  I=0  D=0  UseFilter=on  N=75  TunerSelectOption=Transfer Function Based (PID Tuner App)  InitialConditionSource=internal  InitialConditionForIntegrator=0  InitialConditionForFilter=0  DifferentiatorICPrevScaledInput=0  ExternalReset=none  TrackingMode=off  Kt=1  LimitOutput=off  SatLimitsSource=internal  UpperSaturationLimit=inf  LowerSaturationLimit=-inf  LinearizeAsGain=on  AntiWindupMode=none  Kb=1  POutMin=[]  POutMax=[]  IOutMin=[]  IOutMax=[]  DOutMin=[]  DOutMax=[]  NOutMin=[]  NOutMax=[]  SumOutMin=[]  SumOutMax=[]  SaturationOutMin=[]  SaturationOutMax=[]  PParamMin=[]  PParamMax=[]  IParamMin=[]  IParamMax=[]  DParamMin=[]  DParamMax=[]  NParamMin=[]  NParamMax=[]  KbParamMin=[]  KbParamMax=[]  KtParamMin=[]  KtParamMax=[]  KbOutMin=[]  KbOutMax=[]  KtOutMin=[]  KtOutMax=[]  IntegratorOutMin=[]  IntegratorOutMax=[]  FilterOutMin=[]  FilterOutMax=[]  SumI1OutMin=[]  SumI1OutMax=[]  SumI2OutMin=[]  SumI2OutMax=[]  SumI3OutMin=[]  SumI3OutMax=[]  SumI4OutMin=[]  SumI4OutMax=[]  SumDOutMin=[]  SumDOutMax=[]  DifferentiatorOutMin=[]  DifferentiatorOutMax=[]  FilterDiffOutCoefMin=[]  FilterDiffOutCoefMax=[]  ReciprocalOutMin=[]  ReciprocalOutMax=[]  SumDenOutMin=[]  SumDenOutMax=[]  SumNumOutMin=[]  SumNumOutMax=[]  DivideOutMin=[]  DivideOutMax=[]  UdiffTsProdOutMin=[]  UdiffTsProdOutMax=[]  NTsProdOutMin=[]  NTsProdOutMax=[]  UintegralTsProdOutMin=[]  UintegralTsProdOutMax=[]  UngainTsProdOutMin=[]  UngainTsProdOutMax=[]  IntegratorContinuousStateAttributes=''  IntegratorStateMustResolveToSignalObject=off  IntegratorRTWStateStorageClass=Auto  FilterContinuousStateAttributes=''  FilterStateMustResolveToSignalObject=off  FilterRTWStateStorageClass=Auto  ParallelPVariant=InternalParameters  IdealPVariant=Disabled  IVariant=InternalParameters  DVariant=InternalParameters  IntegratorVariant=Continuous  SatVariant=Disabled  AWVariant=Passthrough  PCopyVariant=Disabled  TRVariant=Disabled  FdbkBlocksVariant=Forward  IdealPFdbkVariant=Disabled  SatFdbkVariant=Disabled  DerivativeFilterVariant=ContFilter  NVariant=InternalParameters  NCopyVariant=Disabled  FilterICVariant=InternalICsFilter  IntegratorICVariant=InternalICs  ExternalResetVariant=Disabled  TRSumVariant=Passthrough  SumFdbkVariant=Disabled  SumVariant=Sum_PID  TsampFilterVariant=InternalTs  TsampNgainVariant=Passthrough  TsampIntegralVariant=Passthrough  ExternalSaturationOutDataTypeStr=Inherit: Same as second input
  Product : Product
  Scope : Scope  NumInputPorts=2
  Scope1 : Scope
  Scope2 : Scope
  Sum : Sum  Inputs=|-+
  To Workspace : ToWorkspace  VariableName=Range_m  SampleTime=-1
  To Workspace1 : ToWorkspace  VariableName=R_commanded  SampleTime=-1
  To Workspace2 : ToWorkspace  VariableName=Error  SampleTime=-1
  stopping_distance : Constant
  Fd : Outport
  wires:
  [R_commanded_m] -> Scope/2
  [Range_m] -> Scope/1
  [Range_m] -> To Workspace/1
  stopping_distance/1 -> Add/2
  [Error] -> Scope1/1
  V_host_mps/1 -> Product/1
  [Error] -> To Workspace2/1
  time_gap_s/1 -> Product/2
  Sum/1 -> [Error], PID Controller/1  "error"
  Add/1 -> [R_commanded_m], Sum/1  "R_commanded_m"
  PID Controller/1 -> Scope2/1, Fd/1
  [R_commanded_m] -> To Workspace1/1
  Range_m/1 -> [Range_m], Sum/2
  Product/1 -> Add/1

== system integrated_controller_scenario3/ACC_control_block/Predictive Speed Assist  ==
  V_limit : Inport
  V_current : Inport  Port=2
  Enable : EnablePort
  MATLAB Function : MATLAB Function  TreatAsAtomicUnit=on
  Scope : Scope
  a_max : Outport
  wires:
  V_limit/1 -> MATLAB Function/1(v_limit)
  V_current/1 -> MATLAB Function/2(v_current)
  MATLAB Function/1(a_max) -> Scope/1, a_max/1

== system integrated_controller_scenario3/ACC_control_block/Velocity_control ==
  V_command : Inport
  V_host : Inport  Port=2
  Enable : EnablePort
  PID Controller : pid_lib/PID Controller  Controller=PID  Form=Parallel  TimeDomain=Continuous-time  UseExternalTs=off  SampleTime=-1  IntegratorMethod=Forward Euler  FilterMethod=Forward Euler  ControllerParametersSource=internal  P=500  I=15  D=0  UseFilter=on  N=75  TunerSelectOption=Transfer Function Based (PID Tuner App)  InitialConditionSource=internal  InitialConditionForIntegrator=0  InitialConditionForFilter=0  DifferentiatorICPrevScaledInput=0  ExternalReset=none  TrackingMode=off  Kt=1  LimitOutput=off  SatLimitsSource=internal  UpperSaturationLimit=inf  LowerSaturationLimit=-inf  LinearizeAsGain=on  AntiWindupMode=none  Kb=1  POutMin=[]  POutMax=[]  IOutMin=[]  IOutMax=[]  DOutMin=[]  DOutMax=[]  NOutMin=[]  NOutMax=[]  SumOutMin=[]  SumOutMax=[]  SaturationOutMin=[]  SaturationOutMax=[]  PParamMin=[]  PParamMax=[]  IParamMin=[]  IParamMax=[]  DParamMin=[]  DParamMax=[]  NParamMin=[]  NParamMax=[]  KbParamMin=[]  KbParamMax=[]  KtParamMin=[]  KtParamMax=[]  KbOutMin=[]  KbOutMax=[]  KtOutMin=[]  KtOutMax=[]  IntegratorOutMin=[]  IntegratorOutMax=[]  FilterOutMin=[]  FilterOutMax=[]  SumI1OutMin=[]  SumI1OutMax=[]  SumI2OutMin=[]  SumI2OutMax=[]  SumI3OutMin=[]  SumI3OutMax=[]  SumI4OutMin=[]  SumI4OutMax=[]  SumDOutMin=[]  SumDOutMax=[]  DifferentiatorOutMin=[]  DifferentiatorOutMax=[]  FilterDiffOutCoefMin=[]  FilterDiffOutCoefMax=[]  ReciprocalOutMin=[]  ReciprocalOutMax=[]  SumDenOutMin=[]  SumDenOutMax=[]  SumNumOutMin=[]  SumNumOutMax=[]  DivideOutMin=[]  DivideOutMax=[]  UdiffTsProdOutMin=[]  UdiffTsProdOutMax=[]  NTsProdOutMin=[]  NTsProdOutMax=[]  UintegralTsProdOutMin=[]  UintegralTsProdOutMax=[]  UngainTsProdOutMin=[]  UngainTsProdOutMax=[]  IntegratorContinuousStateAttributes=''  IntegratorStateMustResolveToSignalObject=off  IntegratorRTWStateStorageClass=Auto  FilterContinuousStateAttributes=''  FilterStateMustResolveToSignalObject=off  FilterRTWStateStorageClass=Auto  ParallelPVariant=InternalParameters  IdealPVariant=Disabled  IVariant=InternalParameters  DVariant=InternalParameters  IntegratorVariant=Continuous  SatVariant=Disabled  AWVariant=Passthrough  PCopyVariant=Disabled  TRVariant=Disabled  FdbkBlocksVariant=Forward  IdealPFdbkVariant=Disabled  SatFdbkVariant=Disabled  DerivativeFilterVariant=ContFilter  NVariant=InternalParameters  NCopyVariant=Disabled  FilterICVariant=InternalICsFilter  IntegratorICVariant=InternalICs  ExternalResetVariant=Disabled  TRSumVariant=Passthrough  SumFdbkVariant=Disabled  SumVariant=Sum_PID  TsampFilterVariant=InternalTs  TsampNgainVariant=Passthrough  TsampIntegralVariant=Passthrough  ExternalSaturationOutDataTypeStr=Inherit: Same as second input
  Scope : Scope  NumInputPorts=2
  Scope1 : Scope
  Sum : Sum  Inputs=|+-
  Fd : Outport
  wires:
  V_command/1 -> Scope/1, Sum/1
  V_host/1 -> Scope/2, Sum/2
  Sum/1 -> PID Controller/1
  PID Controller/1 -> Scope1/1, Fd/1

== system integrated_controller_scenario3/ACC_control_block/manual_mode ==
  Throttle : Inport
  Enable : EnablePort
  Fd : Outport
  wires:
  Throttle/1 -> Fd/1

== system integrated_controller_scenario3/Control Layer/If Action Subsystem ==
  Action Port : ActionPort  ActionPortLabel=if((u1 ==1) & (u2 ==0))
  Constant : Constant  Value=0
  Out1 : Outport
  wires:
  Constant/1 -> Out1/1

== system integrated_controller_scenario3/Control Layer/If Action Subsystem1 ==
  Action Port : ActionPort  ActionPortLabel=else
  Constant : Constant
  Out1 : Outport
  wires:
  Constant/1 -> Out1/1

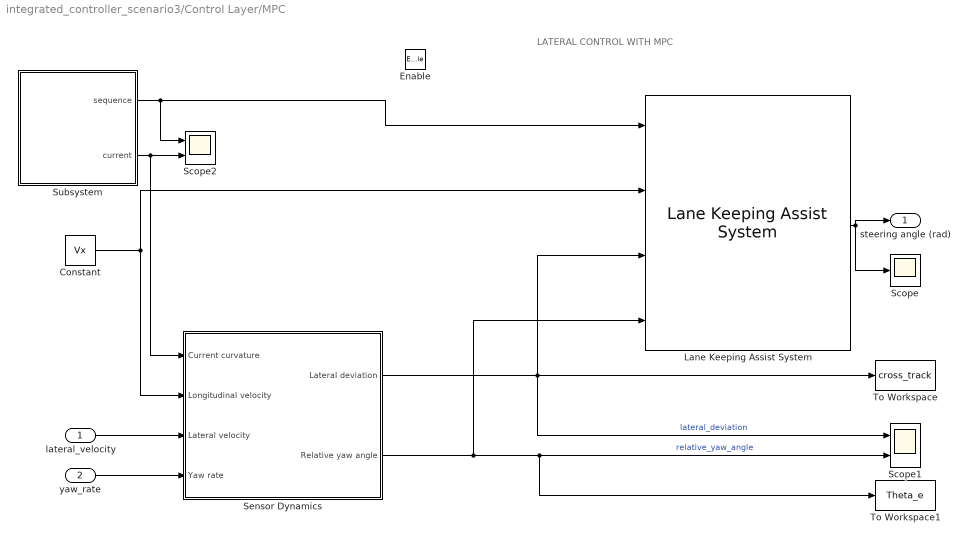
== system integrated_controller_scenario3/Control Layer/MPC ==
  note: LATERAL CONTROL WITH MPC
  lateral_velocity : Inport
  yaw_rate : Inport  Port=2
  Enable : EnablePort
  Constant : Constant  Value=Vx
  Lane Keeping Assist System : mpcadaslib/Lane Keeping Assist System  ModelType=Use vehicle parameters  VehicleMass=1140  VehicleYawInertia=1436.24  LengthToFront=1.165  LengthToRear=1.165  FrontTireStiffness=155494.663  RearTireStiffness=1554494.663  EgoModelMatrixA=[-4.4021 ,-12.4603;1.3913,-5.1868]  EgoModelMatrixB=[24.1270;15.8609]  EgoModelMatrixC=[1,0;0,1]  InitialLongVel=Vx  TransportLag=0  MinSteering=-0.5  umin_ext=off  MaxSteering=0.5  umax_ext=off  Ts=0.1  PredictionHorizon=10  ControllerBehavior=0.500  suboptimal=off  maxiter=10  datatypeopt=double  optmode=off  trackmode=off
      settings: SourceProductBaseCode=MP
  Scope : Scope
  Scope1 : Scope  NumInputPorts=2
  Scope2 : Scope  NumInputPorts=2
  Sensor Dynamics : Subsystem
  Subsystem : Subsystem  mask{signal=md, ts=Ts, steps=10}
      mask prompts: signal "Signal name"; ts "Sampling time"; steps "Number of previewing steps"
      mask init:
      | ts = evalin('base',get_param(gcbh,'ts'));
      | signal = evalin('base',get_param(gcbh,'signal'));
      | steps = evalin('base',get_param(gcbh,'steps'));
      | data = mpc_previewer_maskinit(signal,ts);
      mask Display:
      | fprintf('Future\nsample\nextractor');
      | port_label('output', 1, 'seq')
      | port_label('output', 2, '@t')
  To Workspace : ToWorkspace  VariableName=cross_track  SampleTime=-1
  To Workspace1 : ToWorkspace  VariableName=Theta_e  SampleTime=-1
  steering angle (rad) : Outport
  wires:
  Constant/1 -> Sensor Dynamics/2(Longitudinal velocity), Lane Keeping Assist System/2
  Subsystem/1(sequence) -> Scope2/1, Lane Keeping Assist System/1
  Lane Keeping Assist System/1 -> steering angle (rad)/1, Scope/1
  lateral_velocity/1 -> Sensor Dynamics/3(Lateral velocity)
  yaw_rate/1 -> Sensor Dynamics/4(Yaw rate)
  Sensor Dynamics/2(Relative yaw angle) -> To Workspace1/1, Scope1/2, Lane Keeping Assist System/4  "relative_yaw_angle"
  Subsystem/2(current) -> Scope2/2, Sensor Dynamics/1(Current curvature)
  Sensor Dynamics/1(Lateral deviation) -> To Workspace/1, Scope1/1, Lane Keeping Assist System/3  "lateral_deviation"

== system integrated_controller_scenario3/Control Layer/Pure Pursuit ==
  note: pure pursuit controller
  state : Inport
  waypoints : Inport  Port=2
  Enable : EnablePort
  Pure-pursuit lateral control : Subsystem
  delta : Outport
  wires:
  Pure-pursuit lateral control/1(delta) -> delta/1
  state/1 -> Pure-pursuit lateral control/1(Posistion state)
  waypoints/1 -> Pure-pursuit lateral control/2(waypoints)

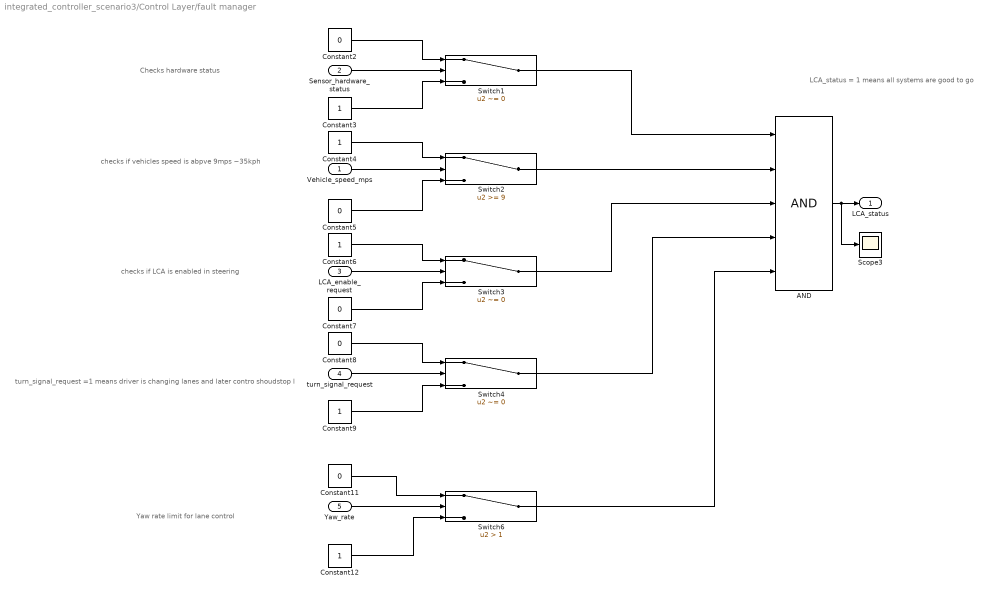
== system integrated_controller_scenario3/Control Layer/fault manager ==
  note: turn_signal_request =1 means driver is changing lanes and later contro shoudstop
      | l
  note: LCA_status = 1 means all systems are good to go
  note: checks if LCA is enabled in steering
  note: checks if vehicles speed is abpve 9mps ~35kph
  note: Checks hardware status
  note: Yaw rate limit for lane control
  Vehicle_speed_mps : Inport
  Sensor_hardware_status : Inport  Port=2
  LCA_enable_request : Inport  Port=3
  turn_signal_request : Inport  Port=4
  Yaw_rate : Inport  Port=5
  AND : Logic  Inputs=5  AllPortsSameDT=off  OutDataTypeStr=boolean
  Constant{2,5,7..8,11} (5 alike) : Constant  Value=0
  Constant{3..4,6,9,12} (5 alike) : Constant
  Scope3 : Scope
  Switch1 : Switch  Criteria=u2 ~= 0
  Switch2 : Switch  Threshold=9
  Switch3 : Switch  Criteria=u2 ~= 0  Threshold=10
  Switch4 : Switch  Criteria=u2 ~= 0  Threshold=10
  Switch6 : Switch  Criteria=u2 > Threshold  Threshold=1
  LCA_status : Outport
  wires:
  Switch1/1 -> AND/1
  Constant9/1 -> Switch4/3
  Switch4/1 -> AND/4
  Constant8/1 -> Switch4/1
  turn_signal_request/1 -> Switch4/2
  Switch3/1 -> AND/3
  Switch2/1 -> AND/2
  Constant7/1 -> Switch3/3
  Constant6/1 -> Switch3/1
  LCA_enable_request/1 -> Switch3/2
  Constant3/1 -> Switch1/3
  Constant2/1 -> Switch1/1
  Constant4/1 -> Switch2/1
  Constant5/1 -> Switch2/3
  Sensor_hardware_status/1 -> Switch1/2
  Vehicle_speed_mps/1 -> Switch2/2
  AND/1 -> Scope3/1, LCA_status/1
  Constant12/1 -> Switch6/3
  Yaw_rate/1 -> Switch6/2
  Constant11/1 -> Switch6/1
  Switch6/1 -> AND/5

== system integrated_controller_scenario3/Control Layer/manual ==
  Enable : EnablePort
  Constant : Constant  Value=0
  delta : Outport
  wires:
  Constant/1 -> delta/1

== system integrated_controller_scenario3/Control Layer/mode manager ==
  LCA_enable : Inport
  road_curvature : Inport  Port=2
  Vehicle_speed : Inport  Port=3
  Chart : Stateflow chart  TreatAsAtomicUnit=on
  Scope : Scope  NumInputPorts=3
  Scope1 : Scope  NumInputPorts=3
  enable_mpc : Outport
  enable_pp : Outport  Port=2
  enable_manual : Outport  Port=3
  wires:
  road_curvature/1 -> Scope1/2, Chart/2(Radius)
  LCA_enable/1 -> Chart/1(LCA_enable), Scope1/1
  Vehicle_speed/1 -> Scope1/3, Chart/3(V_mps)
  Chart/1(en_MPC) -> Scope/1, enable_mpc/1
  Chart/2(en_PP) -> Scope/2, enable_pp/1
  Chart/3(en_man) -> Scope/3, enable_manual/1

== system integrated_controller_scenario3/Input Block/Signal Builder ==
  Demux : Demux  Tag=STV Demux  Outputs=1
      settings: DisplayOption=none
  FromWs : FromWorkspace  Tag=STV FromWs  VariableName=tuvar
      SigBuilderData=|
      | common.afterFinalStr = 'Extrapolate'
      | common.sampleTime = 0
      | dataSet.timeRange = [0 500]
      | dataSet.name = 'Group 1'
      | sbobj.Groups.Name = 'Group 1'
      | sbobj.Groups.Signals.Name = 'ACC_Enable_1'
      | sbobj.Groups.Signals.XData = [0 500]
      | sbobj.Groups.Signals.YData = [1 1]
      | sbobj.Groups.TimeRange = [0 500]
  ACC_Enable_1 : Outport  Tag=STV Outport
  wires:
  FromWs/1 -> Demux/1
  Demux/1 -> ACC_Enable_1/1

== system integrated_controller_scenario3/Input layer/LCA_enable_request_signal ==
  Demux : Demux  Tag=STV Demux  Outputs=1
      settings: DisplayOption=none
  FromWs : FromWorkspace  Tag=STV FromWs  VariableName=tuvar
      SigBuilderData=|
      | common.afterFinalStr = 'Extrapolate'
      | common.sampleTime = 0
      | dataSet.timeRange = [0 10]
      | dataSet.name = 'Group 1'
      | sbobj.Groups.Name = 'Group 1'
      | sbobj.Groups.Signals.Name = 'Signal 2'
      | sbobj.Groups.Signals.XData = [0 10]
      | sbobj.Groups.Signals.YData = [1 1]
  Signal 2 : Outport  Tag=STV Outport
  wires:
  FromWs/1 -> Demux/1
  Demux/1 -> Signal 2/1

== system integrated_controller_scenario3/Input layer/Reference for PP ==
  Constant3 : Constant  Value=xRef  SampleTime=0.1
  Constant4 : Constant  Value=yRef  SampleTime=0.1
  Matrix Concatenate : Concatenate  Mode=Multidimensional array  ConcatenateDimension=2
  Scope : Scope
  Waypoints : Outport
  wires:
  Constant3/1 -> Matrix Concatenate/1
  Constant4/1 -> Scope/1, Matrix Concatenate/2
  Matrix Concatenate/1 -> Waypoints/1

== system integrated_controller_scenario3/Input layer/Road_radius_signal ==
  Demux : Demux  Tag=STV Demux  Outputs=1
      settings: DisplayOption=none
  FromWs : FromWorkspace  Tag=STV FromWs  VariableName=tuvar
      SigBuilderData=|
      | common.afterFinalStr = 'Extrapolate'
      | common.sampleTime = 0
      | dataSet.timeRange = [0 10]
      | dataSet.name = 'Group 1'
      | sbobj.Groups.Name = 'Group 1'
      | sbobj.Groups.Signals.Name = 'Signal 2'
      | sbobj.Groups.Signals.XData = [0 10]
      | sbobj.Groups.Signals.YData = [1 1]
  Signal 2 : Outport  Tag=STV Outport
  wires:
  Demux/1 -> Signal 2/1
  FromWs/1 -> Demux/1

== system integrated_controller_scenario3/Input layer/sensor fault status ==
  Demux : Demux  Tag=STV Demux  Outputs=1
      settings: DisplayOption=none
  FromWs : FromWorkspace  Tag=STV FromWs  VariableName=tuvar
      SigBuilderData=|
      | common.afterFinalStr = 'Extrapolate'
      | common.sampleTime = 0
      | dataSet.timeRange = [0 10]
      | dataSet.name = 'Group 1'
      | sbobj.Groups.Name = 'Group 1'
      | sbobj.Groups.Signals.Name = 'Signal 1'
      | sbobj.Groups.Signals.XData = [0 4 6 10]
      | sbobj.Groups.Signals.YData = [0 0 0 0]
  Signal 1 : Outport  Tag=STV Outport
  wires:
  Demux/1 -> Signal 1/1
  FromWs/1 -> Demux/1

== system integrated_controller_scenario3/Input layer/steering_torque_signal ==
  Demux : Demux  Tag=STV Demux  Outputs=1
      settings: DisplayOption=none
  FromWs : FromWorkspace  Tag=STV FromWs  VariableName=tuvar
      SigBuilderData=|
      | common.afterFinalStr = 'Extrapolate'
      | common.sampleTime = 0
      | dataSet.timeRange = [0 10]
      | dataSet.name = 'Group 1'
      | sbobj.Groups.Name = 'Group 1'
      | sbobj.Groups.Signals.Name = 'Signal 1'
      | sbobj.Groups.Signals.XData = [0 4 6 10]
      | sbobj.Groups.Signals.YData = [0 0 0 0]
  Signal 1 : Outport  Tag=STV Outport
  wires:
  FromWs/1 -> Demux/1
  Demux/1 -> Signal 1/1

== system integrated_controller_scenario3/Input layer/turn_signal ==
  Demux : Demux  Tag=STV Demux  Outputs=1
      settings: DisplayOption=none
  FromWs : FromWorkspace  Tag=STV FromWs  VariableName=tuvar
      SigBuilderData=|
      | common.afterFinalStr = 'Extrapolate'
      | common.sampleTime = 0
      | dataSet.timeRange = [0 10]
      | dataSet.name = 'Group 1'
      | sbobj.Groups.Name = 'Group 1'
      | sbobj.Groups.Signals.Name = 'Signal 2'
      | sbobj.Groups.Signals.XData = [0 10]
      | sbobj.Groups.Signals.YData = [0 0]
  Signal 2 : Outport  Tag=STV Outport
  wires:
  Demux/1 -> Signal 2/1
  FromWs/1 -> Demux/1

== system integrated_controller_scenario3/Radar_sensor_output/If Action Subsystem ==
  Action Port : ActionPort  ActionPortLabel=if(u1 > u2)
  Constant : Constant  Value=0
  Out1 : Outport
  wires:
  Constant/1 -> Out1/1

== system integrated_controller_scenario3/Radar_sensor_output/If Action Subsystem1 ==
  Action Port : ActionPort  ActionPortLabel=else
  Constant : Constant
  Out1 : Outport
  wires:
  Constant/1 -> Out1/1

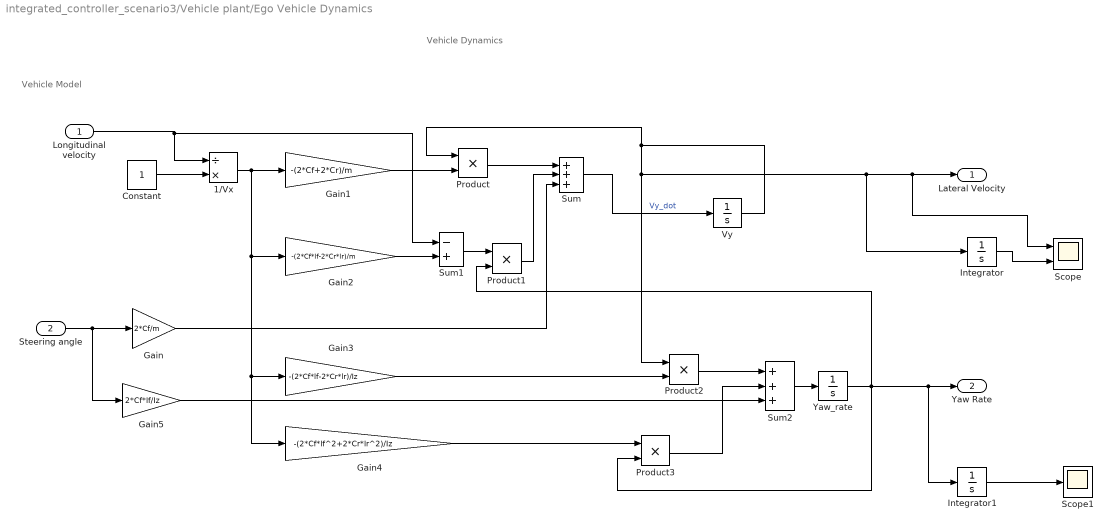
== system integrated_controller_scenario3/Vehicle plant/Ego Vehicle Dynamics ==
  note: Vehicle Model
  note: Vehicle Dynamics
  Longitudinal velocity : Inport
  Steering angle : Inport  Port=2
  1/Vx : Product  Inputs=/*
  Constant : Constant
  Gain : Gain  Gain=2*Cf/m
  Gain1 : Gain  Gain=-(2*Cf+2*Cr)/m
  Gain2 : Gain  Gain=-(2*Cf*lf-2*Cr*lr)/m
  Gain3 : Gain  Gain=-(2*Cf*lf-2*Cr*lr)/Iz
  Gain4 : Gain  Gain=-(2*Cf*lf^2+2*Cr*lr^2)/Iz
  Gain5 : Gain  Gain=2*Cf*lf/Iz
  Integrator : Integrator
  Integrator1 : Integrator
  Product{,1..3} (4 alike) : Product
  Scope : Scope  NumInputPorts=2
  Scope1 : Scope
  Sum : Sum  Inputs=+++
  Sum1 : Sum  Inputs=-+
  Sum2 : Sum  Inputs=+++
  Vy : Integrator
  "Yaw_rate " : Integrator
  Lateral Velocity : Outport  VectorParamsAs1DForOutWhenUnconnected=off
  Yaw Rate : Outport  Port=2  VectorParamsAs1DForOutWhenUnconnected=off
  wires:
  Sum2/1 -> "Yaw_rate "/1
  Gain2/1 -> Sum1/2
  Gain4/1 -> Product3/1
  Constant/1 -> 1/Vx/2
  Gain3/1 -> Product2/2
  1/Vx/1 -> Gain4/1, Gain3/1, Gain2/1, Gain1/1
  Product2/1 -> Sum2/1
  Product3/1 -> Sum2/2
  Gain5/1 -> Sum2/3
  Sum1/1 -> Product1/1
  "Yaw_rate "/1 -> Product3/2, Integrator1/1, Yaw Rate/1, Product1/2
  Gain/1 -> Sum/3
  Steering angle/1 -> Gain/1, Gain5/1
  Gain1/1 -> Product/2
  Product/1 -> Sum/1
  Vy/1 -> Product/1, Integrator/1, Scope/1, Lateral Velocity/1, Product2/1
  Sum/1 -> Vy/1  "Vy_dot"
  Longitudinal velocity/1 -> Sum1/1, 1/Vx/1
  Product1/1 -> Sum/2
  Integrator/1 -> Scope/2
  Integrator1/1 -> Scope1/1

== system integrated_controller_scenario3/Vehicle plant/If Action Subsystem ==
  note: for MPC feedback
  Steering Angle : Inport
  Action Port : ActionPort  ActionPortLabel=if(u1 == 0)
  steering angle to ego dynamics : Outport
  wires:
  Steering Angle/1 -> steering angle to ego dynamics/1

== system integrated_controller_scenario3/Vehicle plant/If Action Subsystem1 ==
  note: for the PP feedback to vehicle dynamics block
  Steering Angle : Inport
  Action Port : ActionPort  ActionPortLabel=else
  wheenangle : Outport
  wires:
  Steering Angle/1 -> wheenangle/1

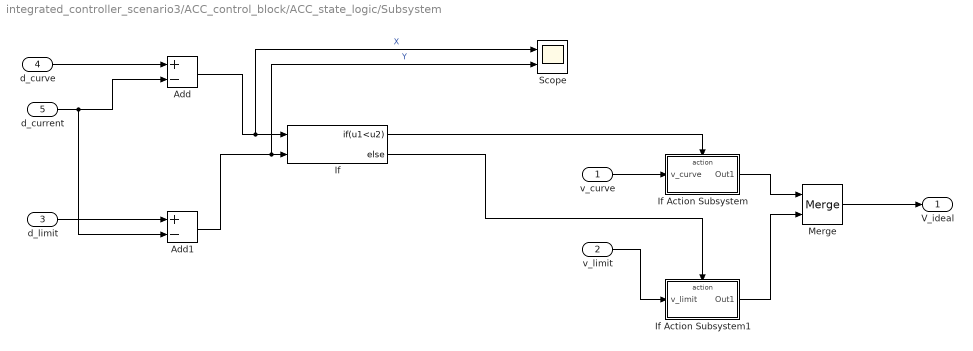
== system integrated_controller_scenario3/ACC_control_block/ACC_state_logic/Subsystem ==
  v_curve : Inport
  v_limit : Inport  Port=2
  d_limit : Inport  Port=3
  d_curve : Inport  Port=4
  d_current : Inport  Port=5
  Add : Sum  Inputs=+-
  Add1 : Sum  Inputs=+-
  If : If  NumInputs=2  IfExpression=u1<u2
  If Action Subsystem : Subsystem  TreatAsAtomicUnit=on
  If Action Subsystem1 : Subsystem  TreatAsAtomicUnit=on
  Merge : Merge
  Scope : Scope  NumInputPorts=2
  V_ideal : Outport
  wires:
  d_limit/1 -> Add1/1
  d_current/1 -> Add1/2, Add/2
  d_curve/1 -> Add/1
  v_curve/1 -> If Action Subsystem/1(v_curve)
  v_limit/1 -> If Action Subsystem1/1(v_limit)
  Add1/1 -> Scope/2, If/2  "Y"
  If/2 -> If Action Subsystem1/Action
  Merge/1 -> V_ideal/1
  If Action Subsystem1/1(Out1) -> Merge/2
  Add/1 -> Scope/1, If/1  "X"
  If/1 -> If Action Subsystem/Action
  If Action Subsystem/1(Out1) -> Merge/1

== system integrated_controller_scenario3/Control Layer/MPC/Sensor Dynamics ==
  Current curvature : Inport
  Longitudinal velocity : Inport  Port=2
  Lateral velocity : Inport  Port=3
  Yaw rate : Inport  Port=4
  Integrator : Integrator
  Integrator2 : Integrator
  Mux1 : Mux  Inputs=[1 1 1]
  Product : Product
  Subtract : Sum  Inputs=-+
  e1dot : Fcn  Expr=u(1)*u(3)+u(2)
  Lateral deviation : Outport  VectorParamsAs1DForOutWhenUnconnected=off
  Relative yaw angle : Outport  Port=2  VectorParamsAs1DForOutWhenUnconnected=off
  wires:
  Current curvature/1 -> Product/2
  Integrator2/1 -> Mux1/3, Relative yaw angle/1  "e2"
  Mux1/1 -> e1dot/1
  e1dot/1 -> Integrator/1
  Longitudinal velocity/1 -> Product/1, Mux1/1
  Lateral velocity/1 -> Mux1/2
  Integrator/1 -> Lateral deviation/1  "e1"
  Product/1 -> Subtract/1
  Yaw rate/1 -> Subtract/2
  Subtract/1 -> Integrator2/1  "e2dot"

== system integrated_controller_scenario3/Control Layer/MPC/Subsystem ==
  MATLAB Function : MATLAB Function  TreatAsAtomicUnit=on
  Memory1 : Memory  InheritSampleTime=on  LinearizeAsDelay=on
  sequence : Outport  VectorParamsAs1DForOutWhenUnconnected=off
  current : Outport  Port=2  VectorParamsAs1DForOutWhenUnconnected=off
  wires:
  MATLAB Function/2(first) -> current/1
  MATLAB Function/3(next_t) -> Memory1/1
  MATLAB Function/1(seq) -> sequence/1
  Memory1/1 -> MATLAB Function/1(t)

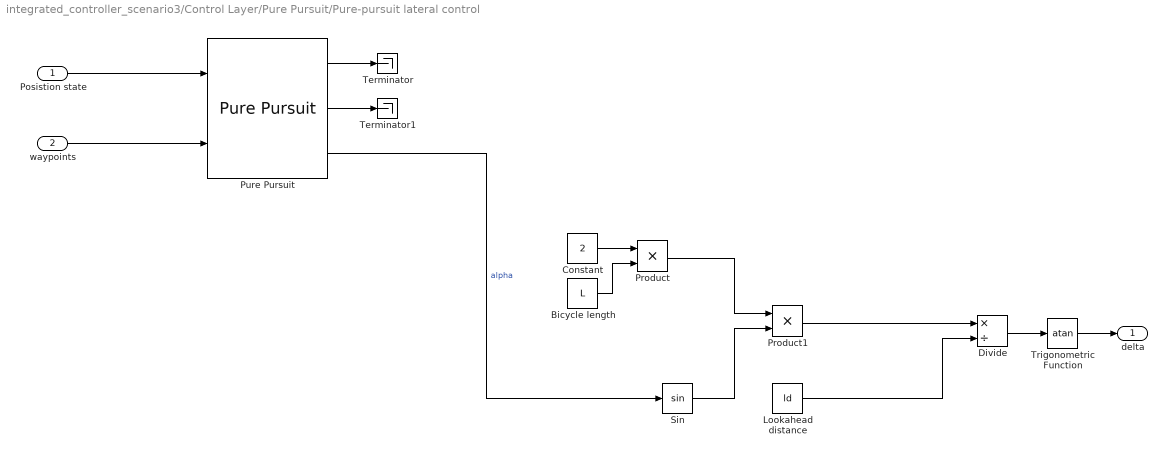
== system integrated_controller_scenario3/Control Layer/Pure Pursuit/Pure-pursuit lateral control ==
  Posistion state : Inport
  waypoints : Inport  Port=2
  Bicycle length : Constant  Value=L
  Constant : Constant  Value=2
  Divide : Product  Inputs=*/
  Lookahead distance : Constant  Value=ld
  Product : Product
  Product1 : Product
  Pure Pursuit : robotalgslib/Pure Pursuit  DesiredLinearVelocity=Vx  MaxAngularVelocity=1.0  LookaheadDistance=ld  TargetDirPort=on  SimulateUsing=Code generation
  Sin : Trigonometry
  Terminator : Terminator
  Terminator1 : Terminator
  Trigonometric Function : Trigonometry  Operator=atan
  delta : Outport
  wires:
  Posistion state/1 -> Pure Pursuit/1
  waypoints/1 -> Pure Pursuit/2
  Pure Pursuit/1 -> Terminator/1
  Pure Pursuit/2 -> Terminator1/1
  Trigonometric Function/1 -> delta/1
  Constant/1 -> Product/1
  Divide/1 -> Trigonometric Function/1
  Lookahead distance/1 -> Divide/2
  Sin/1 -> Product1/2
  Product1/1 -> Divide/1
  Pure Pursuit/3 -> Sin/1  "alpha"
  Bicycle length/1 -> Product/2
  Product/1 -> Product1/1

== system integrated_controller_scenario3/ACC_control_block/ACC_state_logic/Subsystem/If Action Subsystem ==
  v_curve : Inport
  Action Port : ActionPort  ActionPortLabel=if(u1<u2)
  Out1 : Outport
  wires:
  v_curve/1 -> Out1/1

== system integrated_controller_scenario3/ACC_control_block/ACC_state_logic/Subsystem/If Action Subsystem1 ==
  v_limit : Inport
  Action Port : ActionPort  ActionPortLabel=else
  Out1 : Outport
  wires:
  v_limit/1 -> Out1/1

== stateflow chart integrated_controller_scenario3/ACC_control_block/ACC_state_logic/ACC_state_control ==
  state Velocity_and_PSA
    state Velocity_control
      entry: en_man = false;
      en_vel =true;
      en_pos=false;
      en_psa = false;
    state PSA
      entry: en_man = false;
      en_vel =false;
      en_pos=false;
      en_psa = true;
    Velocity_control -> PSA : [v_ideal<v_set]
    (default) -> Velocity_control
    PSA -> Velocity_control : [v_ideal>v_set]
  state Manual_mode
    entry: en_man = true;
    en_vel =false;
    en_pos=false;
  state Headway_control
    entry: en_man = false;
    en_vel =false;
    en_pos=true;
  Manual_mode -> Velocity_and_PSA [order 1] : [(ACC_enable ==1)&&(target_flag==0)]
  Velocity_and_PSA -> Headway_control [order 2] : [(ACC_enable == 1)&(target_flag == 1)&&after(30,sec)]
  Manual_mode -> Headway_control [order 2] : [(ACC_enable == 1) && (target_flag == 1)]
  (default) -> Manual_mode
  Velocity_and_PSA -> Manual_mode [order 1] : [ACC_enable == 0]
  Headway_control -> Velocity_and_PSA [order 2] : [((ACC_enable == 1)&(target_flag==0)|| V_host>commanded_speed + 0.5)&&after(20,sec)]
  Headway_control -> Manual_mode [order 1] : [ACC_enable ==0]
  data: ACC_enable input; V_host input; commanded_speed input; target_flag input; en_man output; en_pos output; en_vel output; en_psa output; v_set input; v_ideal input

== matlab function integrated_controller_scenario3/ACC_control_block/Predictive Speed Assist /MATLAB Function ==
  data: v_limit input; a_max output; v_current input
function a_max = fcn(v_limit,v_current)

if v_current < v_limit+0.2
    a_max = 2000; %mpss
elseif v_current>v_limit+0.2
    a_max = -2000 ; %mpss
else 
    a_max = 0;
    
end

== matlab function integrated_controller_scenario3/Control Layer/MPC/Subsystem/MATLAB Function ==
  settings: updateMethod=DISCRETE  sampleTime=ts
  data: data parameter; seq output; steps parameter; t input; first output; next_t output
function [seq,first,next_t] = fcn(data,steps,t)
%#codegen
[seq,first,next_t] = mpcblock_preview('md',data,steps,t);

== stateflow chart integrated_controller_scenario3/Control Layer/mode manager/Chart ==
  state LCA_off
    entry: en_man = true;
    en_PP = false;
    en_MPC = false;
  state LCA_On
    state PP
      entry: en_man = false;
      en_PP = true;
      en_MPC = false;
    state MPC
      entry: en_man = false;
      en_PP = false;
      en_MPC = true;
    (default) -> PP
    MPC -> PP : [((V_mps <=0.00010) && (Radius >=1000)) ||((V_mps <=0.00010) && (Radius<1000)) ]
    PP -> MPC : [((V_mps >0.00010) && (Radius >=1000)) ||((V_mps >0.00010) && (Radius<1000)) ]
  (default) -> LCA_off
  LCA_On -> LCA_off : [(LCA_enable ==0)]
  LCA_off -> LCA_On : [(LCA_enable ==1)]
  data: LCA_enable input; Radius input; V_mps input; en_MPC output; en_PP output; en_man output
